simulink model "lab_3"  (R2024b)
settings: Solver=VariableStepAuto  StartTime=0.0  StopTime=20  RelTol=1e-3
values from neighbouring files (symbols this model uses):
  d0 = 44.752    [lab_3_data.m]
  d1 = 1    [lab_3_data.m]
  k1 = -2.0530    (= -2.053)    [lab_3_data.m]
  K2 = 0.0609    [lab_3_data.m]
  K3 = 0.2632/K2    (= 4.32183908046)    [lab_3_data.m]
  n0 = -225.747    [lab_3_data.m]
  n1 = -2.598    [lab_3_data.m]
  T_sq = 20    [lab_3_data.m]
  tau = 0.02367    [lab_3_data.m]
undefined symbols (not defined in the file or in its folder): C3_den, C3_num
libraries: cstblocks x3
settings Model: Creator=ishraqanwar  LastModifiedBy=ishraqanwar

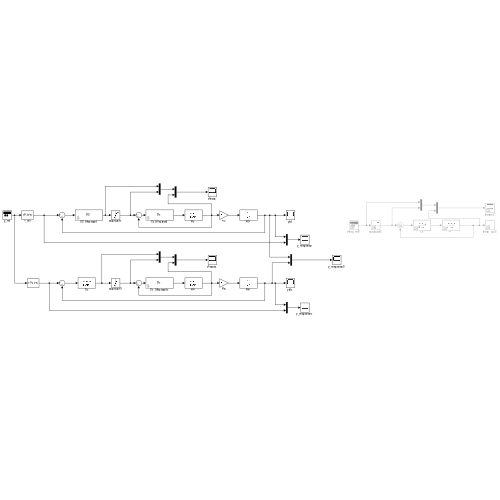
[thumbnail: Simulink's stored preview of the top-level diagram]
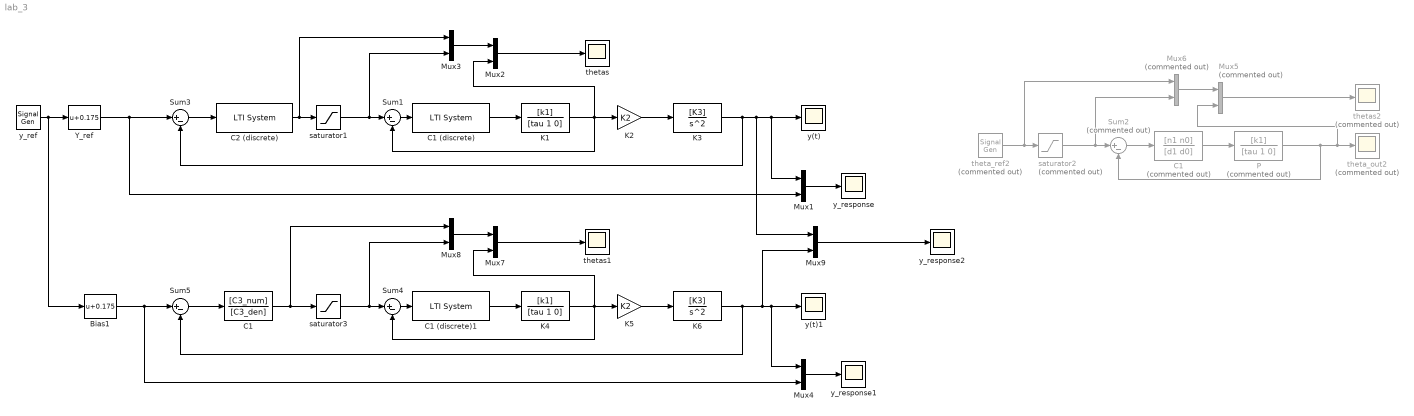
== system lab_3 ==
  " C1" : TransferFcn  Numerator=[C3_num]  Denominator=[C3_den]
  Bias1 : Bias  Bias=0.175  SaturateOnIntegerOverflow=off
  C1 : TransferFcn  Commented=on  Numerator=[n1 n0]  Denominator=[d1 d0]
  C1 (discrete) : cstblocks/LTI System  sys=D1  IC=[]  PadeOrder=0
  C1 (discrete)1 : cstblocks/LTI System  sys=D1  IC=[]  PadeOrder=0
  C2 (discrete) : cstblocks/LTI System  sys=D2  IC=[]  PadeOrder=0
  K1 : TransferFcn  Numerator=[k1]  Denominator=[tau 1 0]
  K2 : Gain  Gain=K2
  K3 : TransferFcn  Numerator=[K3]  Denominator=[1 0 0]
  K4 : TransferFcn  Numerator=[k1]  Denominator=[tau 1 0]
  K5 : Gain  Gain=K2
  K6 : TransferFcn  Numerator=[K3]  Denominator=[1 0 0]
  Mux{1..4,7..9} (7 alike) : Mux  Inputs=2
  Mux5 : Mux  Commented=on  Inputs=2
  Mux6 : Mux  Commented=on  Inputs=2
  P : TransferFcn  Commented=on  Numerator=[k1]  Denominator=[tau 1 0]
  Sum{1,3..5} (4 alike) : Sum  Inputs=|+-
  Sum2 : Sum  Commented=on  Inputs=|+-
  Y_ref : Bias  Bias=0.175  SaturateOnIntegerOverflow=off
  saturator1 : Saturate  UpperLimit=0.7  LowerLimit=-0.7
  saturator2 : Saturate  Commented=on  UpperLimit=0.7  LowerLimit=-0.7
  saturator3 : Saturate  UpperLimit=0.7  LowerLimit=-0.7
  theta_out2 : Scope  Commented=on
  theta_ref2 : SignalGenerator  Commented=on  WaveForm=square  Amplitude=1.0  Frequency=0.5
  thetas : Scope
  thetas1 : Scope
  thetas2 : Scope  Commented=on
  y(t) : Scope
  y(t)1 : Scope
  y_ref : SignalGenerator  WaveForm=square  Amplitude=0.075  Frequency=1/T_sq
  y_response : Scope
  y_response1 : Scope
  y_response2 : Scope
  wires:
  K1/1 -> K2/1, Mux2/2, Sum1/2
  Mux3/1 -> Mux2/1
  Mux2/1 -> thetas/1
  saturator1/1 -> Mux3/2, Sum1/1
  Sum1/1 -> C1 (discrete)/1
  C1 (discrete)/1 -> K1/1
  C1/1 -> P/1
  Mux5/1 -> thetas2/1
  Mux6/1 -> Mux5/1
  saturator2/1 -> Mux6/2, Sum2/1
  theta_ref2/1 -> Mux6/1, saturator2/1
  P/1 -> Sum2/2, Mux5/2, theta_out2/1
  Sum2/1 -> C1/1
  K2/1 -> K3/1
  K3/1 -> Sum3/2, Mux9/1, Mux1/1, y(t)/1
  y_ref/1 -> Bias1/1, Y_ref/1
  Y_ref/1 -> Mux1/2, Sum3/1
  Mux1/1 -> y_response/1
  Sum4/1 -> C1 (discrete)1/1
  C1 (discrete)1/1 -> K4/1
  K4/1 -> K5/1, Mux7/2, Sum4/2
  Mux8/1 -> Mux7/1
  Mux7/1 -> thetas1/1
  saturator3/1 -> Mux8/2, Sum4/1
  Mux4/1 -> y_response1/1
  " C1"/1 -> Mux8/1, saturator3/1
  K5/1 -> K6/1
  Sum5/1 -> " C1"/1
  K6/1 -> Sum5/2, Mux9/2, Mux4/1, y(t)1/1
  Mux9/1 -> y_response2/1
  Bias1/1 -> Mux4/2, Sum5/1
  C2 (discrete)/1 -> Mux3/1, saturator1/1
  Sum3/1 -> C2 (discrete)/1
